simulink model "SatelliteOpticalNetwork_4_projection_v3"  (R2026a)
settings: Solver=ode3  StopTime=cfg.T  FixedStep=cfg.dt
model workspace (MAT data in the model file):
  cfg.n = 4
  cfg.topology = 'mesh'
  cfg.seed = 101
  cfg.dt = 0.02
  cfg.T = 10
  cfg.J = 0.002
  cfg.b = 0.004
  cfg.tau = 0.08
  cfg.umax = 2e-06
  cfg.rateMax = 0.00012
  cfg.lambda = 8
  cfg.K = 8e-05
  cfg.phi = 8e-06
  cfg.kp = 64
  cfg.kd = 14
  cfg.ki = 8
  cfg.initialAngle = [2e-06; -1e-06]
  cfg.noise = 8e-08
  cfg.powerNoise = 0.008
  cfg.Pt = 0.5
  cfg.eta = 0.4
  cfg.divergence = 2e-05
  cfg.aperture = 0.1
  cfg.distance = 800000
  cfg.sensitivity = 1.5e-06
  cfg.capacity = 1000000000
  cfg.offered = 600000000
  cfg.packetBits = 12000
  cfg.c = 299792458
  cfg.processing = 0.0001
  cfg.method = 'proposed'
  cfg.controller = 'SMC'
  cfg.scenario = 'pointing'
  cfg.faultStart = 2
  cfg.faultEnd = 8
  cfg.profile = 'sudden'
  cfg.severity = 1
  cfg.probeAmplitude = 6e-06
  cfg.probeDwell = 0.5
  cfg.maxCorrection = 3.5e-05
  cfg.detectRatio = 0.72
  cfg.decisionPeriod = 0.1
  cfg.warmup = 1
  cfg.edges = [1  2; 1  3; 1  4; 2  3; 3  4]
  cfg.m = 5
  cfg.version = '1.0.0'
  cfg.assumptions = 'Fixed sparse graph; one effective two-axis terminal per bidirectional edge; fluid single flow 1 to 2; no orbital propagation or atmospheric loss.'
  cfg.noiseSamples = [0.0535121228343 0.398971857605 -3.13116194418 0.785317147926 -0.646255228153 0.891855797063 0.932023533057 -1.5355153092 0.0745919923426 -0.661062844199 -0.294971205653 0.972557875124 ... (12625 elements, 505x5x5)]
undefined symbols (not defined in the file or in its folder): terminal_parameters
settings Model: Creator=rishi  LastModifiedBy=kaush

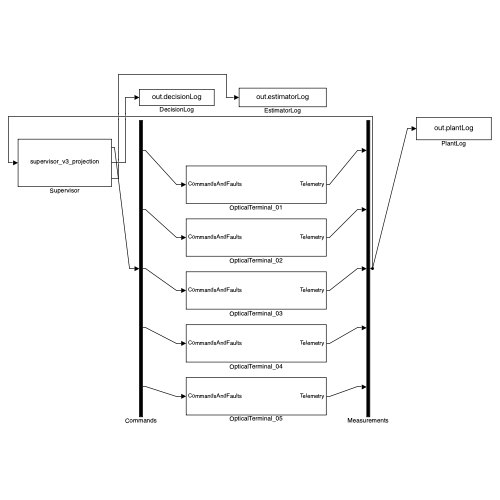
[thumbnail: Simulink's stored preview of the top-level diagram]
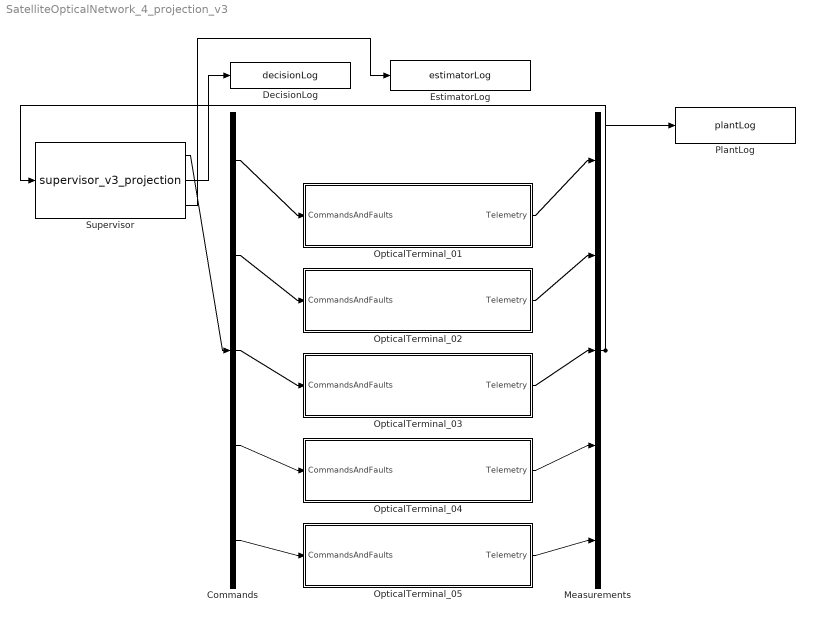
== system SatelliteOpticalNetwork_4_projection_v3 ==
  Commands : Demux  Outputs=[11 11 11 11 11]
  DecisionLog : ToWorkspace  VariableName=decisionLog  SaveFormat=Timeseries  SampleTime=-1
  EstimatorLog : ToWorkspace  VariableName=estimatorLog  SaveFormat=Timeseries  SampleTime=-1
  Measurements : Mux  Inputs=5
  OpticalTerminal_01 : Subsystem
  OpticalTerminal_02 : Subsystem
  OpticalTerminal_03 : Subsystem
  OpticalTerminal_04 : Subsystem
  OpticalTerminal_05 : Subsystem
  PlantLog : ToWorkspace  VariableName=plantLog  SaveFormat=Timeseries  SampleTime=-1
  Supervisor : M-S-Function  FunctionName=supervisor_v3_projection  Parameters=cfg
  wires:
  Supervisor/1 -> Commands/1
  Commands/1 -> OpticalTerminal_01/1(CommandsAndFaults)
  OpticalTerminal_01/1(Telemetry) -> Measurements/1
  Commands/2 -> OpticalTerminal_02/1(CommandsAndFaults)
  OpticalTerminal_02/1(Telemetry) -> Measurements/2
  Commands/3 -> OpticalTerminal_03/1(CommandsAndFaults)
  OpticalTerminal_03/1(Telemetry) -> Measurements/3
  Commands/4 -> OpticalTerminal_04/1(CommandsAndFaults)
  OpticalTerminal_04/1(Telemetry) -> Measurements/4
  Commands/5 -> OpticalTerminal_05/1(CommandsAndFaults)
  OpticalTerminal_05/1(Telemetry) -> Measurements/5
  Measurements/1 -> Supervisor/1, PlantLog/1
  Supervisor/2 -> DecisionLog/1
  Supervisor/3 -> EstimatorLog/1

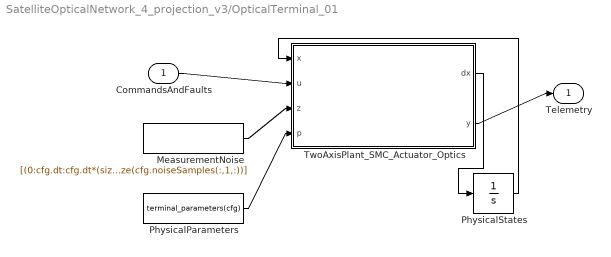
== system SatelliteOpticalNetwork_4_projection_v3/OpticalTerminal_01 ==
  CommandsAndFaults : Inport
  MeasurementNoise : FromWorkspace  VariableName=[(0:cfg.dt:cfg.dt*(size(cfg.noiseSamples,1)-1))' squeeze(cfg.noiseSamples(:,1,:))]  Interpolate=off  OutputAfterFinalValue=Holding final value
  PhysicalParameters : Constant  Value=terminal_parameters(cfg)
  PhysicalStates : Integrator  InitialCondition=[cfg.initialAngle;zeros(6,1)]
  TwoAxisPlant_SMC_Actuator_Optics : MATLAB Function  TreatAsAtomicUnit=on
  Telemetry : Outport
  wires:
  CommandsAndFaults/1 -> TwoAxisPlant_SMC_Actuator_Optics/2(u)
  PhysicalStates/1 -> TwoAxisPlant_SMC_Actuator_Optics/1(x)
  MeasurementNoise/1 -> TwoAxisPlant_SMC_Actuator_Optics/3(z)
  PhysicalParameters/1 -> TwoAxisPlant_SMC_Actuator_Optics/4(p)
  TwoAxisPlant_SMC_Actuator_Optics/1(dx) -> PhysicalStates/1
  TwoAxisPlant_SMC_Actuator_Optics/2(y) -> Telemetry/1

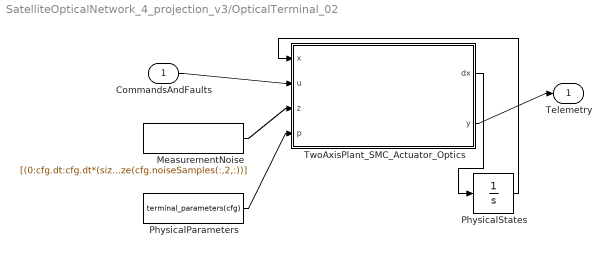
== system SatelliteOpticalNetwork_4_projection_v3/OpticalTerminal_02 ==
  CommandsAndFaults : Inport
  MeasurementNoise : FromWorkspace  VariableName=[(0:cfg.dt:cfg.dt*(size(cfg.noiseSamples,1)-1))' squeeze(cfg.noiseSamples(:,2,:))]  Interpolate=off  OutputAfterFinalValue=Holding final value
  PhysicalParameters : Constant  Value=terminal_parameters(cfg)
  PhysicalStates : Integrator  InitialCondition=[cfg.initialAngle;zeros(6,1)]
  TwoAxisPlant_SMC_Actuator_Optics : MATLAB Function  TreatAsAtomicUnit=on
  Telemetry : Outport
  wires:
  CommandsAndFaults/1 -> TwoAxisPlant_SMC_Actuator_Optics/2(u)
  PhysicalStates/1 -> TwoAxisPlant_SMC_Actuator_Optics/1(x)
  MeasurementNoise/1 -> TwoAxisPlant_SMC_Actuator_Optics/3(z)
  PhysicalParameters/1 -> TwoAxisPlant_SMC_Actuator_Optics/4(p)
  TwoAxisPlant_SMC_Actuator_Optics/1(dx) -> PhysicalStates/1
  TwoAxisPlant_SMC_Actuator_Optics/2(y) -> Telemetry/1

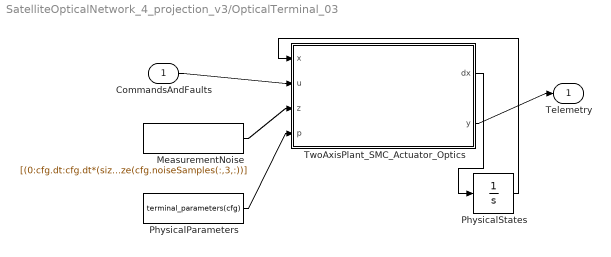
== system SatelliteOpticalNetwork_4_projection_v3/OpticalTerminal_03 ==
  CommandsAndFaults : Inport
  MeasurementNoise : FromWorkspace  VariableName=[(0:cfg.dt:cfg.dt*(size(cfg.noiseSamples,1)-1))' squeeze(cfg.noiseSamples(:,3,:))]  Interpolate=off  OutputAfterFinalValue=Holding final value
  PhysicalParameters : Constant  Value=terminal_parameters(cfg)
  PhysicalStates : Integrator  InitialCondition=[cfg.initialAngle;zeros(6,1)]
  TwoAxisPlant_SMC_Actuator_Optics : MATLAB Function  TreatAsAtomicUnit=on
  Telemetry : Outport
  wires:
  CommandsAndFaults/1 -> TwoAxisPlant_SMC_Actuator_Optics/2(u)
  PhysicalStates/1 -> TwoAxisPlant_SMC_Actuator_Optics/1(x)
  MeasurementNoise/1 -> TwoAxisPlant_SMC_Actuator_Optics/3(z)
  PhysicalParameters/1 -> TwoAxisPlant_SMC_Actuator_Optics/4(p)
  TwoAxisPlant_SMC_Actuator_Optics/1(dx) -> PhysicalStates/1
  TwoAxisPlant_SMC_Actuator_Optics/2(y) -> Telemetry/1

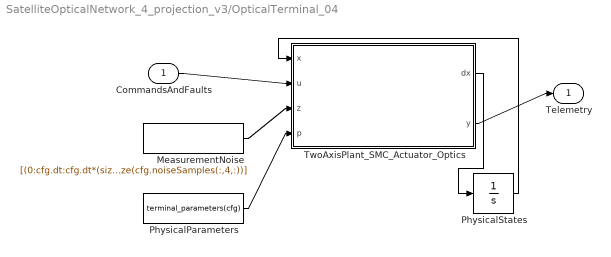
== system SatelliteOpticalNetwork_4_projection_v3/OpticalTerminal_04 ==
  CommandsAndFaults : Inport
  MeasurementNoise : FromWorkspace  VariableName=[(0:cfg.dt:cfg.dt*(size(cfg.noiseSamples,1)-1))' squeeze(cfg.noiseSamples(:,4,:))]  Interpolate=off  OutputAfterFinalValue=Holding final value
  PhysicalParameters : Constant  Value=terminal_parameters(cfg)
  PhysicalStates : Integrator  InitialCondition=[cfg.initialAngle;zeros(6,1)]
  TwoAxisPlant_SMC_Actuator_Optics : MATLAB Function  TreatAsAtomicUnit=on
  Telemetry : Outport
  wires:
  CommandsAndFaults/1 -> TwoAxisPlant_SMC_Actuator_Optics/2(u)
  PhysicalStates/1 -> TwoAxisPlant_SMC_Actuator_Optics/1(x)
  MeasurementNoise/1 -> TwoAxisPlant_SMC_Actuator_Optics/3(z)
  PhysicalParameters/1 -> TwoAxisPlant_SMC_Actuator_Optics/4(p)
  TwoAxisPlant_SMC_Actuator_Optics/1(dx) -> PhysicalStates/1
  TwoAxisPlant_SMC_Actuator_Optics/2(y) -> Telemetry/1

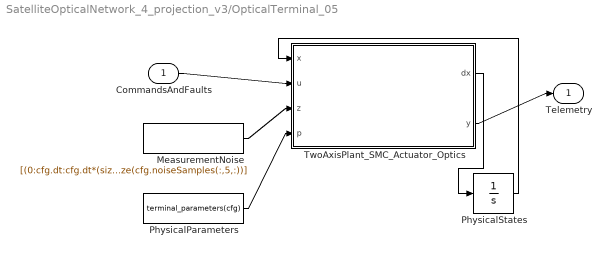
== system SatelliteOpticalNetwork_4_projection_v3/OpticalTerminal_05 ==
  CommandsAndFaults : Inport
  MeasurementNoise : FromWorkspace  VariableName=[(0:cfg.dt:cfg.dt*(size(cfg.noiseSamples,1)-1))' squeeze(cfg.noiseSamples(:,5,:))]  Interpolate=off  OutputAfterFinalValue=Holding final value
  PhysicalParameters : Constant  Value=terminal_parameters(cfg)
  PhysicalStates : Integrator  InitialCondition=[cfg.initialAngle;zeros(6,1)]
  TwoAxisPlant_SMC_Actuator_Optics : MATLAB Function  TreatAsAtomicUnit=on
  Telemetry : Outport
  wires:
  CommandsAndFaults/1 -> TwoAxisPlant_SMC_Actuator_Optics/2(u)
  PhysicalStates/1 -> TwoAxisPlant_SMC_Actuator_Optics/1(x)
  MeasurementNoise/1 -> TwoAxisPlant_SMC_Actuator_Optics/3(z)
  PhysicalParameters/1 -> TwoAxisPlant_SMC_Actuator_Optics/4(p)
  TwoAxisPlant_SMC_Actuator_Optics/1(dx) -> PhysicalStates/1
  TwoAxisPlant_SMC_Actuator_Optics/2(y) -> Telemetry/1

== matlab function SatelliteOpticalNetwork_4_projection_v3/OpticalTerminal_02/TwoAxisPlant_SMC_Actuator_Optics ==
  data: x input; dx output; u input; y output; z input; p input
function [dx,y]=terminal_kernel(x,u,z,p)
%#codegen
J=p(1);b=p(2);tau=p(3);umax=p(4);vmax=p(5);
theta=x(1:2);v=x(3:4);a=x(5:6);r=u(1:2);
ym=theta+u(7:8)+p(13)*u(11)*z(1:2);vm=v+p(13)*2*z(3:4);
e=ym-r;s=vm+p(6)*e;
if p(15)>0
 raw=J*(-p(9)*e-p(10)*vm-p(11)*x(7:8))+b*vm;
else
 raw=b*vm-J*p(6)*vm-J*p(7)*max(-1,min(1,s/p(8)));
end
cmd=max(-umax,min(umax,raw));
dv=(a-b*v)/J;
for k=1:2
 if abs(v(k))>=vmax && sign(v(k))*dv(k)>0,dv(k)=0;end
end
di=e;for k=1:2,if abs(raw(k))>umax,di(k)=0;end,end
dx=[max(-vmax,min(vmax,v));dv;(u(3)*cmd-a)/(tau*u(4));di];
err=theta+u(9:10);
power=p(12)*exp(-2*sum(err.^2)/p(16)^2)*max(0,u(5))*double(u(6)<=0);
q=power/p(17);pm=max(0,power*(1+p(14)*z(5)));
y=[r;theta;err;v;s;cmd;a;double(any(abs(raw)>umax));power;q;double(q>=1);ym;vm;pm;u(3);u(4);u(5)];
end

== matlab function SatelliteOpticalNetwork_4_projection_v3/OpticalTerminal_01/TwoAxisPlant_SMC_Actuator_Optics ==
  data: x input; dx output; u input; y output; z input; p input
function [dx,y]=terminal_kernel(x,u,z,p)
%#codegen
J=p(1);b=p(2);tau=p(3);umax=p(4);vmax=p(5);
theta=x(1:2);v=x(3:4);a=x(5:6);r=u(1:2);
ym=theta+u(7:8)+p(13)*u(11)*z(1:2);vm=v+p(13)*2*z(3:4);
e=ym-r;s=vm+p(6)*e;
if p(15)>0
 raw=J*(-p(9)*e-p(10)*vm-p(11)*x(7:8))+b*vm;
else
 raw=b*vm-J*p(6)*vm-J*p(7)*max(-1,min(1,s/p(8)));
end
cmd=max(-umax,min(umax,raw));
dv=(a-b*v)/J;
for k=1:2
 if abs(v(k))>=vmax && sign(v(k))*dv(k)>0,dv(k)=0;end
end
di=e;for k=1:2,if abs(raw(k))>umax,di(k)=0;end,end
dx=[max(-vmax,min(vmax,v));dv;(u(3)*cmd-a)/(tau*u(4));di];
err=theta+u(9:10);
power=p(12)*exp(-2*sum(err.^2)/p(16)^2)*max(0,u(5))*double(u(6)<=0);
q=power/p(17);pm=max(0,power*(1+p(14)*z(5)));
y=[r;theta;err;v;s;cmd;a;double(any(abs(raw)>umax));power;q;double(q>=1);ym;vm;pm;u(3);u(4);u(5)];
end

== matlab function SatelliteOpticalNetwork_4_projection_v3/OpticalTerminal_03/TwoAxisPlant_SMC_Actuator_Optics ==
  data: x input; dx output; u input; y output; z input; p input
function [dx,y]=terminal_kernel(x,u,z,p)
%#codegen
J=p(1);b=p(2);tau=p(3);umax=p(4);vmax=p(5);
theta=x(1:2);v=x(3:4);a=x(5:6);r=u(1:2);
ym=theta+u(7:8)+p(13)*u(11)*z(1:2);vm=v+p(13)*2*z(3:4);
e=ym-r;s=vm+p(6)*e;
if p(15)>0
 raw=J*(-p(9)*e-p(10)*vm-p(11)*x(7:8))+b*vm;
else
 raw=b*vm-J*p(6)*vm-J*p(7)*max(-1,min(1,s/p(8)));
end
cmd=max(-umax,min(umax,raw));
dv=(a-b*v)/J;
for k=1:2
 if abs(v(k))>=vmax && sign(v(k))*dv(k)>0,dv(k)=0;end
end
di=e;for k=1:2,if abs(raw(k))>umax,di(k)=0;end,end
dx=[max(-vmax,min(vmax,v));dv;(u(3)*cmd-a)/(tau*u(4));di];
err=theta+u(9:10);
power=p(12)*exp(-2*sum(err.^2)/p(16)^2)*max(0,u(5))*double(u(6)<=0);
q=power/p(17);pm=max(0,power*(1+p(14)*z(5)));
y=[r;theta;err;v;s;cmd;a;double(any(abs(raw)>umax));power;q;double(q>=1);ym;vm;pm;u(3);u(4);u(5)];
end

== matlab function SatelliteOpticalNetwork_4_projection_v3/OpticalTerminal_04/TwoAxisPlant_SMC_Actuator_Optics ==
  data: x input; dx output; u input; y output; z input; p input
function [dx,y]=terminal_kernel(x,u,z,p)
%#codegen
J=p(1);b=p(2);tau=p(3);umax=p(4);vmax=p(5);
theta=x(1:2);v=x(3:4);a=x(5:6);r=u(1:2);
ym=theta+u(7:8)+p(13)*u(11)*z(1:2);vm=v+p(13)*2*z(3:4);
e=ym-r;s=vm+p(6)*e;
if p(15)>0
 raw=J*(-p(9)*e-p(10)*vm-p(11)*x(7:8))+b*vm;
else
 raw=b*vm-J*p(6)*vm-J*p(7)*max(-1,min(1,s/p(8)));
end
cmd=max(-umax,min(umax,raw));
dv=(a-b*v)/J;
for k=1:2
 if abs(v(k))>=vmax && sign(v(k))*dv(k)>0,dv(k)=0;end
end
di=e;for k=1:2,if abs(raw(k))>umax,di(k)=0;end,end
dx=[max(-vmax,min(vmax,v));dv;(u(3)*cmd-a)/(tau*u(4));di];
err=theta+u(9:10);
power=p(12)*exp(-2*sum(err.^2)/p(16)^2)*max(0,u(5))*double(u(6)<=0);
q=power/p(17);pm=max(0,power*(1+p(14)*z(5)));
y=[r;theta;err;v;s;cmd;a;double(any(abs(raw)>umax));power;q;double(q>=1);ym;vm;pm;u(3);u(4);u(5)];
end

== matlab function SatelliteOpticalNetwork_4_projection_v3/OpticalTerminal_05/TwoAxisPlant_SMC_Actuator_Optics ==
  data: x input; dx output; u input; y output; z input; p input
function [dx,y]=terminal_kernel(x,u,z,p)
%#codegen
J=p(1);b=p(2);tau=p(3);umax=p(4);vmax=p(5);
theta=x(1:2);v=x(3:4);a=x(5:6);r=u(1:2);
ym=theta+u(7:8)+p(13)*u(11)*z(1:2);vm=v+p(13)*2*z(3:4);
e=ym-r;s=vm+p(6)*e;
if p(15)>0
 raw=J*(-p(9)*e-p(10)*vm-p(11)*x(7:8))+b*vm;
else
 raw=b*vm-J*p(6)*vm-J*p(7)*max(-1,min(1,s/p(8)));
end
cmd=max(-umax,min(umax,raw));
dv=(a-b*v)/J;
for k=1:2
 if abs(v(k))>=vmax && sign(v(k))*dv(k)>0,dv(k)=0;end
end
di=e;for k=1:2,if abs(raw(k))>umax,di(k)=0;end,end
dx=[max(-vmax,min(vmax,v));dv;(u(3)*cmd-a)/(tau*u(4));di];
err=theta+u(9:10);
power=p(12)*exp(-2*sum(err.^2)/p(16)^2)*max(0,u(5))*double(u(6)<=0);
q=power/p(17);pm=max(0,power*(1+p(14)*z(5)));
y=[r;theta;err;v;s;cmd;a;double(any(abs(raw)>umax));power;q;double(q>=1);ym;vm;pm;u(3);u(4);u(5)];
end
